simulink model "TScanner2023a"  (R2023a)
settings: Solver=ode4  StartTime=0.0  StopTime=10.0  FixedStep=0.01  RelTol=1e-3
libraries: AFCToolbox x4
settings Model: Creator=zqinghua  LastModifiedBy=zqhkd
settings OptimizationCC: DefaultParameterBehavior=Inlined  EnhancedBackFolding=on  PassReuseOutputArgsAs=Individual arguments  ZeroExternalMemoryAtStartup=off  ZeroInternalMemoryAtStartup=off  OptimizeBlockOrder=speed  DifferentSizesBufferReuse=on  OptimizationCustomize=off  EfficientTunableParamExpr=on
settings DebuggingCC: ParameterTunabilityLossMsg=error
settings HardwareCC: ProdBitPerInt=16  ProdBitPerPointer=16  ProdBitPerSizeT=16  ProdBitPerPtrDiffT=16  ProdLargestAtomicFloat=None  ProdWordSize=16  ProdHWDeviceType=STMicroelectronics->ST10/Super10
settings SFSimCC: MATLABDynamicMemAlloc=off
settings RTWCC: Description=Embedded Coder  SystemTargetFile=AFCHawk.tlc  GenCodeOnly=on  TemplateMakefile=ert_default_tmf
settings CodeAppCC: ForceParamTrailComments=on  IgnoreCustomStorageClasses=off  OperatorAnnotations=on  SimulinkDataObjDesc=on  SFDataObjDesc=on  InsertBlockDesc=on
settings STFCustomTargetCC: MultiwordLength=256  ModelReferenceCompliant=off  ConcurrentExecutionCompliant=off  CombineOutputUpdateFcns=on  ERTCustomFileBanners=on  SupportContinuousTime=off  SupportNonInlinedSFcns=off  RemoveResetFunc=on  MATLABClassNameForMDSCustomization=Simulink.SoftwareTarget.ERTCustomization  GRTInterface=off  UseToolchainInfoCompliant=off  SystemTargetFile=AFCHawk.tlc
settings ERTTargetCC: TargetLangStandard=C99 (ISO)  ModelReferenceCompliant=off  ParMdlRefBuildCompliant=off  CompOptLevelCompliant=off  ConcurrentExecutionCompliant=off  ModelStepFunctionPrototypeControlCompliant=off  CPPClassGenCompliant=off  UseToolchainInfoCompliant=off  InlinedParameterPlacement=NonHierarchical  ERTCustomFileTemplate=example_file_process.tlc
settings ConfigComp: CovBoundaryAbsTol=1.0e-5

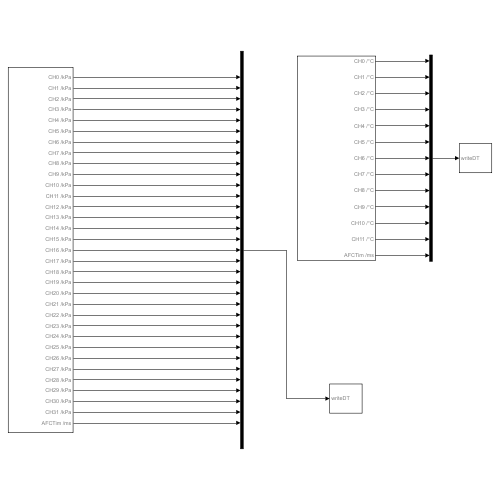
[thumbnail: Simulink's stored preview of the top-level diagram]
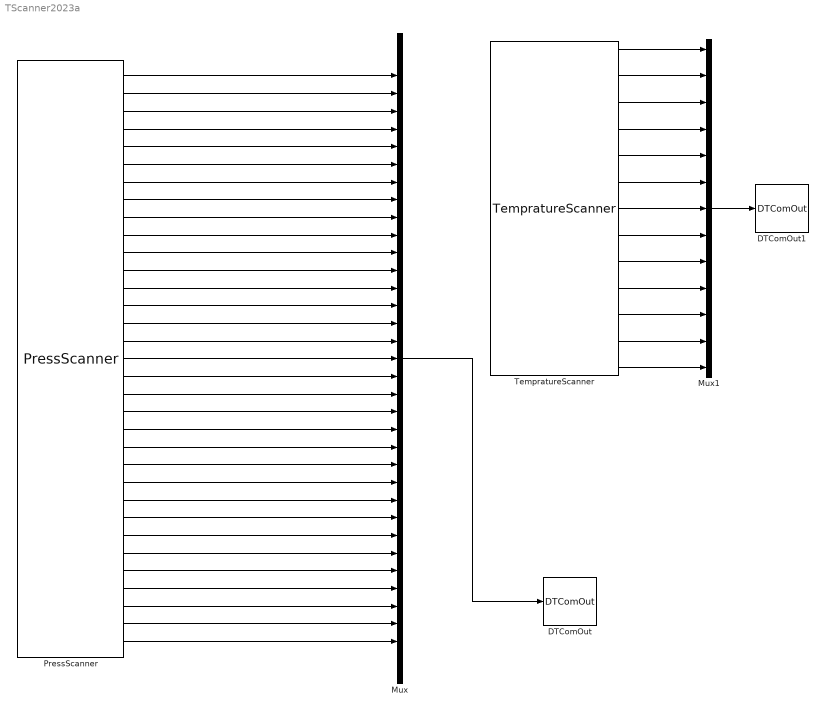
== system TScanner2023a ==
  DTComOut : AFCToolbox/DeviceModule/DTComOut  Priority=8  g_frameType=5  g_outFreq=1  g_comPort=0  g_instName=0  g_id=0
      settings: SourceProductName=AFCToolbox
  DTComOut1 : AFCToolbox/DeviceModule/DTComOut  Priority=8  g_frameType=1  g_outFreq=1  g_comPort=0  g_instName=0  g_id=0
      settings: SourceProductName=AFCToolbox
  Mux : Mux  Inputs=33
  Mux1 : Mux  Inputs=13
  PressScanner : AFCToolbox/DeviceModule/PressScanner  Priority=1  g_sampleTime=0.1  g_comPort=6  g_instName=0  g_id=0
      settings: SourceProductName=AFCToolbox
  TempratureScanner : AFCToolbox/DeviceModule/TempratureScanner  Priority=1  g_sampleTime=0.1  g_comPort=6  g_instName=0  g_id=0
      settings: SourceProductName=AFCToolbox
  wires:
  PressScanner/1 -> Mux/1
  PressScanner/2 -> Mux/2
  PressScanner/3 -> Mux/3
  PressScanner/4 -> Mux/4
  PressScanner/5 -> Mux/5
  PressScanner/6 -> Mux/6
  PressScanner/7 -> Mux/7
  PressScanner/8 -> Mux/8
  PressScanner/9 -> Mux/9
  PressScanner/10 -> Mux/10
  PressScanner/11 -> Mux/11
  PressScanner/12 -> Mux/12
  PressScanner/13 -> Mux/13
  PressScanner/14 -> Mux/14
  PressScanner/15 -> Mux/15
  PressScanner/16 -> Mux/16
  PressScanner/17 -> Mux/17
  PressScanner/18 -> Mux/18
  PressScanner/19 -> Mux/19
  PressScanner/20 -> Mux/20
  PressScanner/21 -> Mux/21
  PressScanner/22 -> Mux/22
  PressScanner/23 -> Mux/23
  PressScanner/24 -> Mux/24
  PressScanner/25 -> Mux/25
  PressScanner/26 -> Mux/26
  PressScanner/27 -> Mux/27
  PressScanner/28 -> Mux/28
  PressScanner/29 -> Mux/29
  PressScanner/30 -> Mux/30
  PressScanner/31 -> Mux/31
  PressScanner/32 -> Mux/32
  PressScanner/33 -> Mux/33
  Mux/1 -> DTComOut/1
  TempratureScanner/1 -> Mux1/1
  TempratureScanner/2 -> Mux1/2
  TempratureScanner/3 -> Mux1/3
  TempratureScanner/4 -> Mux1/4
  TempratureScanner/5 -> Mux1/5
  TempratureScanner/6 -> Mux1/6
  TempratureScanner/7 -> Mux1/7
  TempratureScanner/8 -> Mux1/8
  TempratureScanner/9 -> Mux1/9
  TempratureScanner/10 -> Mux1/10
  TempratureScanner/11 -> Mux1/11
  TempratureScanner/12 -> Mux1/12
  TempratureScanner/13 -> Mux1/13
  Mux1/1 -> DTComOut1/1
